simulink model "library"  (R2026b)
settings: Solver=VariableStepAuto
libraries: hdlsllib x2, simulink x1
settings Model: Creator=guion  LastModifiedBy=guion

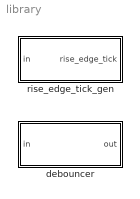
== system library ==
  debouncer : Subsystem
  rise_edge_tick_gen : Subsystem

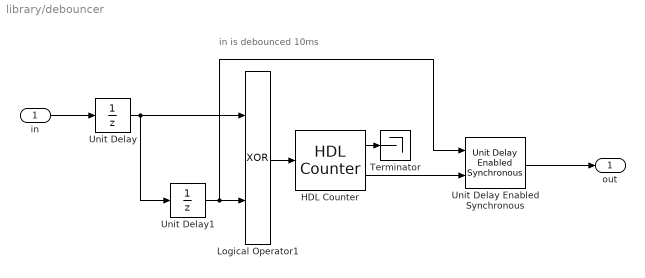
== system library/debouncer ==
  note: in is debounced 10ms
  in : Inport
  HDL Counter : hdlsllib/Sources/HDL Counter  CountType=Count limited  CountInit=0  CountStep=1  CountMax=500000  CountFromType=Initial value  CountFrom=0  CountResetPort=on  CountLoadPort=off  CountEnbPort=off  CountDirPort=off  CountHitOutputPort=on  CountDataType=Unsigned  CountWordLen=19  CountFracLen=0  CountSampTime=1
  Logical Operator1 : Logic  Operator=XOR  AllPortsSameDT=off  OutDataTypeStr=boolean
  Terminator : Terminator
  Unit Delay : UnitDelay  SampleTime=-1
  Unit Delay Enabled Synchronous : hdlsllib/Discrete/Unit Delay Enabled Synchronous  InitialCondition=0.0  SampleTime=-1
  Unit Delay1 : UnitDelay  SampleTime=-1
  out : Outport
  wires:
  in/1 -> Unit Delay/1
  Unit Delay/1 -> Unit Delay1/1, Logical Operator1/1
  Unit Delay1/1 -> Unit Delay Enabled Synchronous/1, Logical Operator1/2
  Logical Operator1/1 -> HDL Counter/1
  Unit Delay Enabled Synchronous/1 -> out/1
  HDL Counter/2 -> Unit Delay Enabled Synchronous/2
  HDL Counter/1 -> Terminator/1

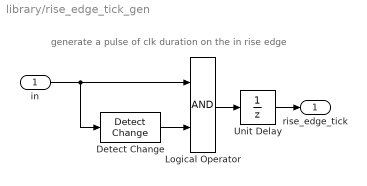
== system library/rise_edge_tick_gen ==
  note: generate a pulse of clk duration on the in rise edge
  in : Inport
  Detect Change : simulink/Logic and Bit Operations/Detect Change  vinit=0  OutDataTypeStr=boolean
      settings: LibrarySourceBlock=|
      | hdlsllib/Logic and Bit
      | Operations/Detect
      | Change
  Logical Operator : Logic  AllPortsSameDT=off  OutDataTypeStr=boolean
  Unit Delay : UnitDelay  SampleTime=-1
  rise_edge_tick : Outport
  wires:
  Logical Operator/1 -> Unit Delay/1
  Detect Change/1 -> Logical Operator/2
  in/1 -> Logical Operator/1, Detect Change/1
  Unit Delay/1 -> rise_edge_tick/1
